simulink model "Stage7_OpenXstimHybrid"  (R2025a)
settings: Solver=FixedStepDiscrete  StartTime=0.0  StopTime=0.008  FixedStep=2.5e-07  RelTol=1e-3
settings Model: Creator=arnav  LastModifiedBy=arnav

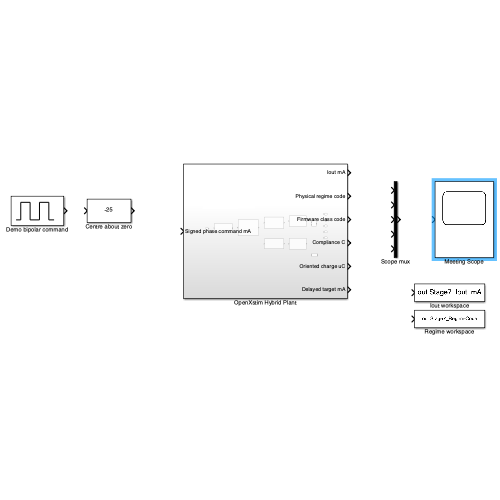
[thumbnail: Simulink's stored preview of the top-level diagram]
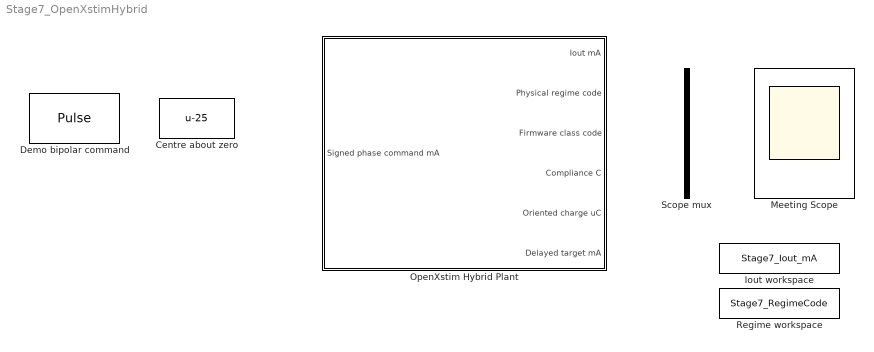
== system Stage7_OpenXstimHybrid ==
  Centre about zero : Bias  Bias=-25  SaturateOnIntegerOverflow=off
  Demo bipolar command : DiscretePulseGenerator  PulseType=Time based  Amplitude=50  Period=0.004  PulseWidth=50  PhaseDelay=0.0005
  Iout workspace : ToWorkspace  VariableName=Stage7_Iout_mA  SaveFormat=Timeseries  SampleTime=-1
  Meeting Scope : Scope
      settings: ActiveDisplayYMinimum=-1  ActiveDisplayYMaximum=1
  OpenXstim Hybrid Plant : Subsystem
  Regime workspace : ToWorkspace  VariableName=Stage7_RegimeCode  SaveFormat=Timeseries  SampleTime=-1
  Scope mux : Mux  Inputs=5

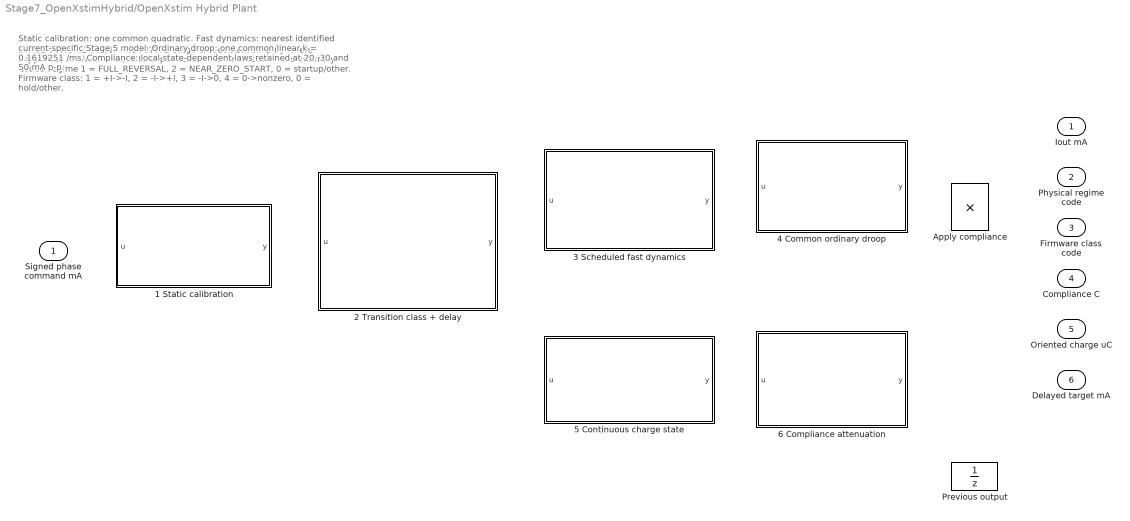
== system Stage7_OpenXstimHybrid/OpenXstim Hybrid Plant ==
  note: STAGE 7 HYBRID PLANT PROTOTYPE
      | Stage 6A decision: simplify where supported, retain current/state dependence where reduction loses accuracy.
      | Codes: regime 1 = FULL_REVERSAL, 2 = NEAR_ZERO_START, 0 = startup/other.
      | Firmware class: 1 = +I->-I, 2 = -I->+I, 3 = -I->0, 4 = 0->nonzero, 0 = hold/other.
  note: Static calibration: one common quadratic.
      | Fast dynamics: nearest identified current-specific Stage 5 model.
      | Ordinary droop: one common linear k = 0.1619251 /ms.
      | Compliance: local state-dependent laws retained at 20, 30 and 50 mA p-p.
  Signed phase command mA : Inport
  1 Static calibration : MATLAB Function  TreatAsAtomicUnit=on
  2 Transition class + delay : MATLAB Function  TreatAsAtomicUnit=on
  3 Scheduled fast dynamics : MATLAB Function  TreatAsAtomicUnit=on
  4 Common ordinary droop : MATLAB Function  TreatAsAtomicUnit=on
  5 Continuous charge state : MATLAB Function  TreatAsAtomicUnit=on
  6 Compliance attenuation : MATLAB Function  TreatAsAtomicUnit=on
  Apply compliance : Product
  Previous output : UnitDelay  SampleTime=2.5e-07  HasFrameUpgradeWarning=on
  Iout mA : Outport
  Physical regime code : Outport  Port=2
  Firmware class code : Outport  Port=3
  Compliance C : Outport  Port=4
  Oriented charge uC : Outport  Port=5
  Delayed target mA : Outport  Port=6

== matlab function Stage7_OpenXstimHybrid/OpenXstim Hybrid Plant/1 Static calibration ==
  data: u input; y output
function y = fcn(u)

y = u;

== matlab function Stage7_OpenXstimHybrid/OpenXstim Hybrid Plant/3 Scheduled fast dynamics ==
  data: u input; y output
function y = fcn(u)

y = u;

== matlab function Stage7_OpenXstimHybrid/OpenXstim Hybrid Plant/4 Common ordinary droop ==
  data: u input; y output
function y = fcn(u)

y = u;

== matlab function Stage7_OpenXstimHybrid/OpenXstim Hybrid Plant/5 Continuous charge state ==
  data: u input; y output
function y = fcn(u)

y = u;

== matlab function Stage7_OpenXstimHybrid/OpenXstim Hybrid Plant/6 Compliance attenuation ==
  data: u input; y output
function y = fcn(u)

y = u;

== matlab function Stage7_OpenXstimHybrid/OpenXstim Hybrid Plant/2 Transition class + delay ==
  data: u input; y output
function y = fcn(u)

y = u;
